simulink model "Copy_of_soft_switch_new_simulation"  (R2025a)
settings: Solver=ode15s  StartTime=0.0  StopTime=0.25  MaxStep=1e-6  RelTol=1e-5
InitFcn:
  | run param_file.m
values from neighbouring files (symbols this model uses):
  param = struct()    [Copy_of_param_file.m]    (also in param_file.m; param_file_loss_vs_freq.m; param_file_original.m; param_file_turbine.m)
settings Model: Creator=user  LastModifiedBy=user

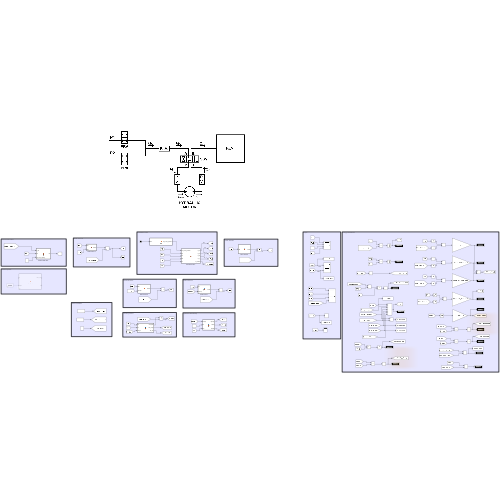
[thumbnail: Simulink's stored preview of the top-level diagram]
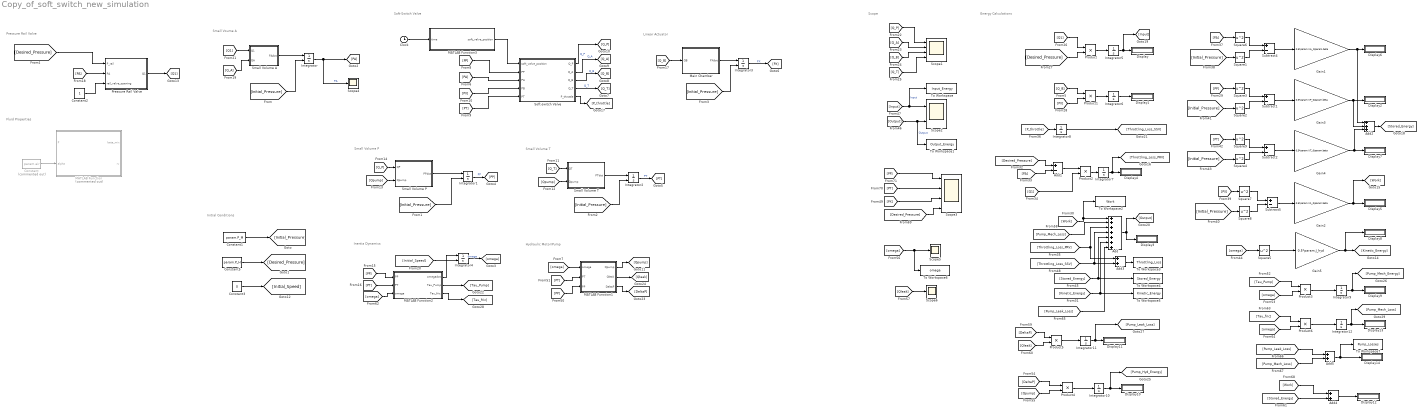
== system Copy_of_soft_switch_new_simulation ==
  note: Fluid Properties
  note: Energy Calculations
  note: Pressure Rail Valve
  note: Scope
  note: Initial Conditions
  note: Small Voume A
  note: Hydraulic Motor/Pump
  note: Inertia Dynamics
  note: Small Volume T
  note: Small Volume P
  note: Soft-Switch Valve
  note: Linear Actuator
  Add : Sum  Inputs=+++++++
  Add1 : Sum  Inputs=+-
  Add2 : Sum  Inputs=+++
  Add3 : Sum
  Add4 : Sum
  Add5 : Sum
  Clock : Clock
  Constant : Constant  Commented=on  Value=param.air
  Constant1 : Constant  Value=param.P_M
  Constant2 : Constant
  Constant3 : Constant  Value=0
  Constant5 : Constant  Value=param.P_H
  Display{,1..14} (15 alike) : Display
  Gain1 : Gain  Gain=0.5*param.VA_0/param.beta
  Gain2 : Gain  Gain=0.5*param.V1_0/param.beta
  Gain3 : Gain  Gain=0.5*param.VP_0/param.beta
  Gain4 : Gain  Gain=0.5*param.VT_0/param.beta
  Gain5 : Gain  Gain=0.5*param.J_hyd
  Integrator{,1..4} (5 alike) : Integrator  InitialConditionSource=external
  Integrator{5..12} (8 alike) : Integrator
  MATLAB Function : MATLAB Function  Commented=on  TreatAsAtomicUnit=on
  MATLAB Function1 : MATLAB Function  TreatAsAtomicUnit=on
  MATLAB Function2 : MATLAB Function  TreatAsAtomicUnit=on
  MATLAB Function3 : MATLAB Function  TreatAsAtomicUnit=on
  Main Chamber : MATLAB Function  TreatAsAtomicUnit=on
  Pressure Rail Valve : MATLAB Function  TreatAsAtomicUnit=on
  Product{,1..6} (7 alike) : Product
  Scope1 : Scope  NumInputPorts=4
      settings: ActiveDisplayYMinimum=-0.00094060960760663083  ActiveDisplayYMaximum=0.00094060960760663083
  Scope2 : Scope  NumInputPorts=2
      settings: ActiveDisplayYMinimum=8.12603993185979  ActiveDisplayYMaximum=8.3876943536714634
  Scope3 : Scope  NumInputPorts=4
      settings: ActiveDisplayYMinimum=2.5851249851028705E+6  ActiveDisplayYMaximum=1.1203875080461368E+7  DataLoggingVariableName=ScopeData2
  Scope4 : Scope
      settings: ActiveDisplayYMinimum=2.5851242431125245E+6  ActiveDisplayYMaximum=1.1203881811987281E+7  DataLoggingVariableName=ScopeData4
  Scope5 : Scope
      settings: ActiveDisplayYMinimum=112.38461410380874  ActiveDisplayYMaximum=113.69317874093653  DataLoggingVariableName=ScopeData3
  Scope6 : Scope
      settings: ActiveDisplayYMinimum=-2.1163885820684094E-7  ActiveDisplayYMaximum=1.4152197079471591E-6  DataLoggingVariableName=ScopeData5
  Small Volume A : MATLAB Function  TreatAsAtomicUnit=on
  Small Volume P : MATLAB Function  TreatAsAtomicUnit=on
  Small Volume T : MATLAB Function  TreatAsAtomicUnit=on
  Soft-switch Valve : MATLAB Function  TreatAsAtomicUnit=on
  Square{1..9} (9 alike) : Math  Operator=square
  Subtract{1..2,4..5} (4 alike) : Sum  Inputs=+-
  To Workspace : ToWorkspace  VariableName=Input_Energy  SaveFormat=Timeseries  SampleTime=-1
  To Workspace1 : ToWorkspace  VariableName=Output_Energy  SaveFormat=Timeseries  SampleTime=-1
  To Workspace2 : ToWorkspace  VariableName=Work  SaveFormat=Timeseries  SampleTime=-1
  To Workspace3 : ToWorkspace  VariableName=Throttling_Loss  SaveFormat=Timeseries  SampleTime=-1
  To Workspace4 : ToWorkspace  VariableName=Stored_Energy  SaveFormat=Timeseries  SampleTime=-1
  To Workspace5 : ToWorkspace  VariableName=Kinetic_Energy  SaveFormat=Timeseries  SampleTime=-1
  To Workspace6 : ToWorkspace  VariableName=omega  SaveFormat=Timeseries  SampleTime=-1
  To Workspace7 : ToWorkspace  VariableName=Pump_Losses  SaveFormat=Timeseries  SampleTime=-1
  wires:
  [Desired_Pressure] -> Pressure Rail Valve/1(P_rail)
  Pressure Rail Valve/1(Q1) -> [Q1]
  Small Volume A/1(PAdot) -> Integrator/1
  Constant1/1 -> [Initial_Pressure]
  [Initial_Pressure] -> Integrator/2
  Integrator/1 -> [PA], Scope4/1  "PA"
  Small Volume P/1(PPdot) -> Integrator1/1
  [Initial_Pressure] -> Integrator1/2
  Small Volume T/1(PTdot) -> Integrator2/1
  [Initial_Pressure] -> Integrator2/2
  Main Chamber/1(PXdot) -> Integrator3/1
  [Initial_Pressure] -> Integrator3/2
  Integrator3/1 -> [PX]  "PX"
  Constant2/1 -> Pressure Rail Valve/3(rail_valve_opening)
  Constant5/1 -> [Desired_Pressure]
  MATLAB Function3/1(soft_valve_position) -> Soft-switch Valve/1(soft_valve_position)
  Clock/1 -> MATLAB Function3/1(time)
  [PA] -> Soft-switch Valve/3(PA)
  [omega] -> MATLAB Function1/1(omega)
  Integrator1/1 -> [PP]  "PP"
  Integrator2/1 -> [PT]  "PT"
  [PP] -> Soft-switch Valve/2(PP)
  [PT] -> Soft-switch Valve/5(PT)
  [PX] -> Soft-switch Valve/4(PB)
  Soft-switch Valve/4(Q_T) -> [Q_T]  "Q_T"
  Soft-switch Valve/3(Q_B) -> [Q_B]  "Q_B"
  Soft-switch Valve/2(Q_A) -> [Q_A]  "Q_A"
  [Q_T] -> Small Volume T/1(QT)
  MATLAB Function1/1(Qpump) -> [Qpump]
  [Qpump] -> Small Volume T/2(Qpump)
  [Qpump] -> Small Volume P/2(Qpump)
  [Q_P] -> Small Volume P/1(QP)
  [Q_B] -> Main Chamber/1(QB)
  [PA] -> Pressure Rail Valve/2(PA)
  [Q_A] -> Small Volume A/2(QA)
  Constant3/1 -> [Initial_Speed]
  [Q1] -> Small Volume A/1(Q1)
  [Q_P] -> Scope1/1
  [Q_A] -> Scope1/2
  [Q_B] -> Scope1/3
  [Q_T] -> Scope1/4
  [Q1] -> Product/1
  [Desired_Pressure] -> Product/2
  Product/1 -> Integrator5/1
  [Q_B] -> Product1/1
  [PX] -> Product1/2
  Product1/1 -> Integrator6/1
  Integrator5/1 -> [Input], Display/1
  Integrator6/1 -> Display1/1
  [Work] -> To Workspace2/1, Add/1
  [Kinetic_Energy] -> To Workspace5/1, Add/6
  Add/1 -> Display3/1, [Output]
  [Desired_Pressure] -> Add1/1
  [PA] -> Add1/2
  Add1/1 -> Product2/1
  [Q1] -> Product2/2
  Product2/1 -> Integrator7/1
  Integrator7/1 -> [Throttling_Loss_PRV], Display4/1
  [Throttling_Loss_PRV] -> Add/3, Add3/1
  Soft-switch Valve/1(Q_P) -> [Q_P]  "Q_P"
  Soft-switch Valve/5(P_throttle) -> [P_throttle]
  [P_throttle] -> Integrator8/1
  [PA] -> Square6/1
  Subtract5/1 -> Gain2/1
  Gain2/1 -> [Work], Display5/1
  Gain1/1 -> Add2/1, Display6/1
  Gain3/1 -> Add2/2, Display2/1
  Gain5/1 -> Display8/1, [Kinetic_Energy]
  Square5/1 -> Gain5/1
  [omega] -> Square5/1
  [Stored_Energy] -> To Workspace4/1, Add/5
  [Initial_Pressure] -> Square1/1
  Square6/1 -> Subtract4/1
  Square1/1 -> Subtract4/2
  [PX] -> Square7/1
  [Initial_Pressure] -> Square8/1
  Subtract4/1 -> Gain1/1
  Square7/1 -> Subtract5/1
  Square8/1 -> Subtract5/2
  Square2/1 -> Subtract1/2
  Square3/1 -> Subtract1/1
  Square9/1 -> Subtract2/1
  Square4/1 -> Subtract2/2
  Subtract2/1 -> Gain4/1
  [PT] -> Square9/1
  [Initial_Pressure] -> Square4/1
  [PP] -> Square3/1
  [Initial_Pressure] -> Square2/1
  Subtract1/1 -> Gain3/1
  Gain4/1 -> Add2/3, Display7/1
  Add2/1 -> [Stored_Energy]
  [Input] -> To Workspace/1, Scope2/1  "Input"
  [Output] -> To Workspace1/1, Scope2/2  "Output"
  Integrator8/1 -> [Throttling_Loss_SSV]
  [Throttling_Loss_SSV] -> Add/4, Add3/2
  Add3/1 -> To Workspace3/1
  [PX] -> Scope3/3
  [PT] -> MATLAB Function2/2(PT)
  MATLAB Function2/2(Tau_Pump) -> [Tau_Pump]
  [PP] -> MATLAB Function2/1(PP)
  [Initial_Speed] -> Integrator4/2
  Integrator4/1 -> [omega]  "omega"
  MATLAB Function2/1(omegadot) -> Integrator4/1
  [omega] -> Product3/2
  [Tau_Pump] -> Product3/1
  Integrator9/1 -> [Pump_Mech_Energy], Display9/1
  Product3/1 -> Integrator9/1
  MATLAB Function1/3(DeltaP) -> [DeltaP]
  [DeltaP] -> Product4/1
  [Qpump] -> Product4/2
  Product4/1 -> Integrator10/1
  Integrator10/1 -> [Pump_Hyd_Energy], Display10/1
  [omega] -> To Workspace6/1, Scope5/1
  MATLAB Function1/2(Qleak) -> [Qleak]
  [Qleak] -> Scope6/1
  [PT] -> MATLAB Function1/2(PT)
  [PP] -> MATLAB Function1/3(PP)
  [DeltaP] -> Product5/1
  [Qleak] -> Product5/2
  Product5/1 -> Integrator11/1
  Integrator11/1 -> [Pump_Leak_Loss], Display11/1
  [Pump_Mech_Loss] -> Add/2
  [omega] -> MATLAB Function2/3(omega)
  MATLAB Function2/3(Tau_fric) -> [Tau_fric]
  [Tau_fric] -> Product6/1
  [omega] -> Product6/2
  Product6/1 -> Integrator12/1
  Integrator12/1 -> [Pump_Mech_Loss], Display13/1
  [Pump_Leak_Loss] -> Add/7
  [Pump_Leak_Loss] -> Add5/1
  [Pump_Mech_Loss] -> Add5/2
  Add5/1 -> To Workspace7/1, Display14/1
  [Work] -> Add4/1
  [Stored_Energy] -> Add4/2
  Add4/1 -> Display12/1
  [Desired_Pressure] -> Scope3/4
  [PT] -> Scope3/2
  [PP] -> Scope3/1
  Constant/1 -> MATLAB Function/2(alpha)

== matlab function Copy_of_soft_switch_new_simulation/MATLAB Function3 ==
  data: time input; soft_valve_position output
function soft_valve_position = fcn(time)

if time > 0.0643
    soft_valve_position = 0;
else
    soft_valve_position = 1;
end

== matlab function Copy_of_soft_switch_new_simulation/MATLAB Function ==
  data: P input; beta_mix output; alpha input; rv output; param parameter
function [beta_mix, rv] = oil_comp(P,alpha,param)
% OIL_COMP compressibility or oil / air mixture
%   beta = spot bulk modulus of mixture at p; [Pa]
%   W = volumetric energy density [J/m^3] 
%   rv = volume ratio

% beta = 1.4e9; 
% %alpha=0.5/100 %0.05%
% alpha = 0;
param.gamma = 1.4;

%Ph=7e6, P0=1e5
Pg=P-P_atmospheric;   % Gauge pressure
r=P/P_atmospheric;    % Pressure ratio
e=exp(Pg/param.beta); 
rv=(1./e+alpha*r.^(-1/param.gamma))/(1+alpha);      %Volume ratio

beta_mix = rv*(1+alpha)/(1/(e*param.beta)+...
           alpha/(param.gamma*P_atmospheric*r^(1/param.gamma+1)));

== matlab function Copy_of_soft_switch_new_simulation/Small Volume A ==
  data: Q1 input; PAdot output; QA input; param parameter
function PAdot = fcn(Q1,QA, param)

PAdot = (param.beta/param.VA_0)*(Q1-QA);

== matlab function Copy_of_soft_switch_new_simulation/Pressure Rail Valve ==
  data: P_rail input; Q1 output; PA input; param parameter; rail_valve_opening input
function Q1 = fcn(P_rail,PA,param,rail_valve_opening)

Q1 = param.Cd*rail_valve_opening*param.max_Avt*sqrt(2/param.rho)...
    *sqrt(abs(P_rail-PA))*sign(P_rail-PA);

== matlab function Copy_of_soft_switch_new_simulation/Soft-switch Valve ==
  data: soft_valve_position input; Q_P output; PP input; PA input; PB input; PT input; Q_A output; Q_B output; Q_T output; param parameter; P_throttle output
function [Q_P, Q_A, Q_B, Q_T, P_throttle] = fcn(soft_valve_position, PP, PA, PB, PT, param)

db = 0.02; % spool deadband around zero (fraction of full stroke)

soft_valve_position = max(-1, min(1, soft_valve_position));

if abs(soft_valve_position) <= db
    f = 0;
else
    f = (abs(soft_valve_position) - db) / (1 - db);
    f = max(0, min(1, f));
end

A_PA = 0; A_PB = 0; A_AT = 0; A_BT = 0; A_PT = 0; A_AB = 0;

if abs(soft_valve_position) <= db
    A_PT = param.max_Avt;
    A_AB = param.max_Avt;
elseif soft_valve_position > 0
    A_PA = param.max_Avt * f;
    A_BT = param.max_Avt * f;
elseif soft_valve_position < 0
    A_PB = param.max_Avt * f;
    A_AT = param.max_Avt * f;
end

Q_PA = param.Cd*A_PA*sign(PP-PA)*sqrt((2/param.rho)*abs(PP-PA));
Q_PB = param.Cd*A_PB*sign(PP-PB)*sqrt((2/param.rho)*abs(PP-PB));
Q_AT = param.Cd*A_AT*sign(PA-PT)*sqrt((2/param.rho)*abs(PA-PT));
Q_BT = param.Cd*A_BT*sign(PB-PT)*sqrt((2/param.rho)*abs(PB-PT));
Q_PT = param.Cd*A_PT*sign(PP-PT)*sqrt((2/param.rho)*abs(PP-PT));
Q_AB = param.Cd*A_AB*sign(PA-PB)*sqrt((2/param.rho)*abs(PA-PB));

Q_P = -(Q_PA + Q_PB + Q_PT);
Q_A =  Q_AT + Q_AB - Q_PA;
Q_B =  Q_BT - Q_AB - Q_PB;
Q_T =  -Q_PT - Q_AT - Q_BT;

Q_B = -Q_B;

P_throttle = ...
    abs(Q_PA)*abs(PP-PA) + ...
    abs(Q_PB)*abs(PP-PB) + ...
    abs(Q_AT)*abs(PA-PT) + ...
    abs(Q_BT)*abs(PB-PT) + ...
    abs(Q_PT)*abs(PP-PT) + ...
    abs(Q_AB)*abs(PA-PB);

end

== matlab function Copy_of_soft_switch_new_simulation/Small Volume P ==
  data: QP input; PPdot output; Qpump input; param parameter
function PPdot = fcn(QP,Qpump, param)

PPdot = (param.beta/param.VP_0)*(QP-Qpump);

== matlab function Copy_of_soft_switch_new_simulation/MATLAB Function1 ==
  data: Qpump output; Qleak output; omega input; PT input; PP input; param parameter; DeltaP output
function [Qpump, Qleak, DeltaP] = fcn(omega, PT, PP, param)
    % Analytical leakage model (Simscape-equivalent)
    
    % Parameters
    D     = param.D;          
    eta_v = param.eta_v_nom;  % nominal volumetric efficiency
    omega_nom = param.omega_nom;      % [rad/s]
    DeltaP_nom = param.dp_nom;    % [Pa]
    rho   = param.rho;        % [kg/m^3]
    
    % Pressure difference
    DeltaP = PP - PT;
    
    % Hagen–Poiseuille coefficient
    K = (D/(2*pi))*omega_nom*(1 - eta_v)/DeltaP_nom;
    
    % Mass leakage flow
    m_dot_leak = K * rho * DeltaP;
    
    % Convert to volumetric leakage
    Qleak = m_dot_leak / rho;
    
    % Ideal displacement flow
    Qideal = (D/(2*pi)) * omega;
    
    % Net flow (same convention as Simscape)
    Qpump = Qideal + Qleak;
end

== matlab function Copy_of_soft_switch_new_simulation/Small Volume T ==
  data: QT input; PTdot output; Qpump input; param parameter
function PTdot = fcn(QT,Qpump,param)

PTdot = (param.beta/param.VT_0)*(Qpump-QT);

== matlab function Copy_of_soft_switch_new_simulation/Main Chamber ==
  data: QB input; PXdot output; param parameter
function PXdot = fcn(QB, param)

PXdot = (param.beta/param.V1_0)*(QB);

== matlab function Copy_of_soft_switch_new_simulation/MATLAB Function2 ==
  data: omegadot output; param parameter; PP input; PT input; Tau_Pump output; omega input; Tau_fric output
function [omegadot, Tau_Pump, Tau_fric] = fcn(param, PP, PT, omega)

dP = PP - PT;

Tau_ideal = (param.D/(2*pi)) * dP;

Tau_fr_nom = ((1 - param.eta_m_nom)/param.eta_m_nom) ...
              * (param.D/(2*pi)) * param.dp_nom;

k = (Tau_fr_nom - param.tau0) / param.dp_nom;

omega_nom_rad = 2*pi*param.omega_nom/60;

s = tanh(4*omega/(5e-5*omega_nom_rad));

Tau_fric = (param.tau0 + k*abs(dP)) * s;

Tau_Pump = Tau_ideal - Tau_fric;

omegadot = Tau_Pump / param.J_hyd;

end
